simulink model "heatdrive_ecc_coupled_se21"  (R2025b)
settings: Solver=ode23t  StartTime=0.0  StopTime=10  FixedStep=0.1  MaxStep=0.4  RelTol=1e-2  AbsTol=1e-3
values from neighbouring files (symbols this model uses):
  cold_load_heat_W = 0.0    (= 0)    [Build_Simulink_Exchange_Params.m]
  cold_load_T_init = get_stage_field(stage_config, 'cold_load_T_in', get_stage_field(stage_config,          'chip_T_in', get_option_field(exchange_options, 'cold_load_T_init', get_option_field(exchange_options, 'chip_T_init', 293.0))))    [Build_Simulink_Exchange_Params.m]    (also in Create_Simulink_Exchange_Runtime.m = get_option_field(options, 'cold_load_T_init',          get_o)
  cold_sink_T_init = get_stage_field(stage_config, 'cold_sink_T_in', get_option_field(exchange_options, 'cold_sink_T_init', 293.0))    [Build_Simulink_Exchange_Params.m]    (also in Create_Simulink_Exchange_Runtime.m = get_option_field(options, 'cold_sink_T_init', ambient_T_init)
  hot_sink_T_init = get_stage_field(stage_config, 'hot_sink_T_in', get_option_field(exchange_options, 'hot_sink_T_init', 293.0))    [Build_Simulink_Exchange_Params.m]    (also in Create_Simulink_Exchange_Runtime.m = get_option_field(options, 'hot_sink_T_init', ambient_T_init))
  mdot_cooldown_source_kgps = mdot_target_kgps    [Build_Simulink_Exchange_Params.m]
  mdot_hold_source_kgps = mdot_target_kgps    [Build_Simulink_Exchange_Params.m]
  pressure_pi_bias_MPa = pressure_pi_dp_guess_MPa    [Build_Simulink_Exchange_Params.m]
  pressure_pi_error_filter_tau_s = max(get_option_field(exchange_options, 'pressure_pi_error_filter_tau_s', 0.002), 1.0e-5)    [Build_Simulink_Exchange_Params.m]
  pressure_pi_error_normalization_gain_kgps_inv = 1.0    (= 1)    [Build_Simulink_Exchange_Params.m]
  pressure_pi_max_MPa = pressure_pi_dp_guess_MPa + pressure_pi_margin_MPa    [Build_Simulink_Exchange_Params.m]
  shex_sink_T_init = get_option_field(exchange_options, 'shex_sink_T_init', hot_sink_T_init)    [Build_Simulink_Exchange_Params.m]
undefined symbols (not defined in the file or in its folder): constitutive_sample_time_s, constitutive_state21_initial, se_constitutive_T21_initial, se_pressure_integrator_max_MPa, se_pressure_pi_ki_MPa_per_kgps_s, se_pressure_pi_kp_MPa_per_kgps, se_pressure_pi_min_MPa, se_solver_T_init_21_internal, se_stage2_pressure_integrator_min_MPa, se_stage4_pressure_integrator_min_MPa, sma_constitutive_T21_initial, sma_mdot_stage1_source_kgps, sma_mdot_stage3_source_kgps, sma_pressure_integrator_max_MPa, sma_pressure_integrator_min_MPa, sma_pressure_pi_ki_MPa_per_kgps_s, sma_pressure_pi_kp_MPa_per_kgps, sma_pressure_pi_min_MPa, sma_solver_T_init_21_internal
libraries: fl_lib x484, nesl_utility x232, SimscapeFluids_lib x20
(part 7 of 8)

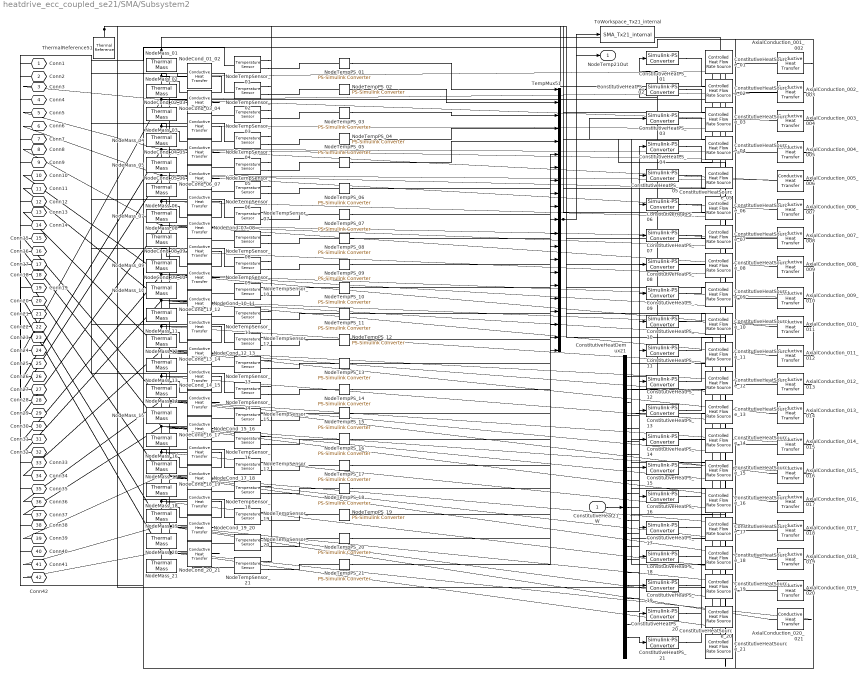
== system heatdrive_ecc_coupled_se21/SMA/Subsystem2 ==
  ConstitutiveHeat21_W : Inport
  AxialConduction_001_002 : fl_lib/Thermal/Thermal Elements/Conductive Heat Transfer  thermal_type=foundation.enum.ConstantVariableTabulated.Constant  wall_geometry=foundation.enum.ConductionWallGeometry.Planar  area=sma_solid_axial_area_m2 m^2  thickness=sma_solid_node_dx_m m  d_in=0.05 m  d_out=0.1 m  L=1 m  th_cond_min=10 W/(K*m)  th_cond=sma_solid_k_W_per_mK W/(K*m)  th_cond_TLU=[413, 401, 392, 383, 371, 357, 342] W/(K*m)  temp_TLU=[200, 273, 400, 600, 800, 1000, 1200] K  T_specify=off  T_priority=None  T=0 K  T_nominal_specify=off  T_nominal_value=1  T_nominal_unit=K  Q_specify=off  Q_priority=None  Q=0 W  Q_nominal_specify=off  Q_nominal_value=1  Q_nominal_unit=W
  AxialConduction_002_003 : fl_lib/Thermal/Thermal Elements/Conductive Heat Transfer  thermal_type=foundation.enum.ConstantVariableTabulated.Constant  wall_geometry=foundation.enum.ConductionWallGeometry.Planar  area=sma_solid_axial_area_m2 m^2  thickness=sma_solid_node_dx_m m  d_in=0.05 m  d_out=0.1 m  L=1 m  th_cond_min=10 W/(K*m)  th_cond=sma_solid_k_W_per_mK W/(K*m)  th_cond_TLU=[413, 401, 392, 383, 371, 357, 342] W/(K*m)  temp_TLU=[200, 273, 400, 600, 800, 1000, 1200] K  T_specify=off  T_priority=None  T=0 K  T_nominal_specify=off  T_nominal_value=1  T_nominal_unit=K  Q_specify=off  Q_priority=None  Q=0 W  Q_nominal_specify=off  Q_nominal_value=1  Q_nominal_unit=W
  AxialConduction_003_004 : fl_lib/Thermal/Thermal Elements/Conductive Heat Transfer  thermal_type=foundation.enum.ConstantVariableTabulated.Constant  wall_geometry=foundation.enum.ConductionWallGeometry.Planar  area=sma_solid_axial_area_m2 m^2  thickness=sma_solid_node_dx_m m  d_in=0.05 m  d_out=0.1 m  L=1 m  th_cond_min=10 W/(K*m)  th_cond=sma_solid_k_W_per_mK W/(K*m)  th_cond_TLU=[413, 401, 392, 383, 371, 357, 342] W/(K*m)  temp_TLU=[200, 273, 400, 600, 800, 1000, 1200] K  T_specify=off  T_priority=None  T=0 K  T_nominal_specify=off  T_nominal_value=1  T_nominal_unit=K  Q_specify=off  Q_priority=None  Q=0 W  Q_nominal_specify=off  Q_nominal_value=1  Q_nominal_unit=W
  AxialConduction_004_005 : fl_lib/Thermal/Thermal Elements/Conductive Heat Transfer  thermal_type=foundation.enum.ConstantVariableTabulated.Constant  wall_geometry=foundation.enum.ConductionWallGeometry.Planar  area=sma_solid_axial_area_m2 m^2  thickness=sma_solid_node_dx_m m  d_in=0.05 m  d_out=0.1 m  L=1 m  th_cond_min=10 W/(K*m)  th_cond=sma_solid_k_W_per_mK W/(K*m)  th_cond_TLU=[413, 401, 392, 383, 371, 357, 342] W/(K*m)  temp_TLU=[200, 273, 400, 600, 800, 1000, 1200] K  T_specify=off  T_priority=None  T=0 K  T_nominal_specify=off  T_nominal_value=1  T_nominal_unit=K  Q_specify=off  Q_priority=None  Q=0 W  Q_nominal_specify=off  Q_nominal_value=1  Q_nominal_unit=W
  AxialConduction_005_006 : fl_lib/Thermal/Thermal Elements/Conductive Heat Transfer  thermal_type=foundation.enum.ConstantVariableTabulated.Constant  wall_geometry=foundation.enum.ConductionWallGeometry.Planar  area=sma_solid_axial_area_m2 m^2  thickness=sma_solid_node_dx_m m  d_in=0.05 m  d_out=0.1 m  L=1 m  th_cond_min=10 W/(K*m)  th_cond=sma_solid_k_W_per_mK W/(K*m)  th_cond_TLU=[413, 401, 392, 383, 371, 357, 342] W/(K*m)  temp_TLU=[200, 273, 400, 600, 800, 1000, 1200] K  T_specify=off  T_priority=None  T=0 K  T_nominal_specify=off  T_nominal_value=1  T_nominal_unit=K  Q_specify=off  Q_priority=None  Q=0 W  Q_nominal_specify=off  Q_nominal_value=1  Q_nominal_unit=W
  AxialConduction_006_007 : fl_lib/Thermal/Thermal Elements/Conductive Heat Transfer  thermal_type=foundation.enum.ConstantVariableTabulated.Constant  wall_geometry=foundation.enum.ConductionWallGeometry.Planar  area=sma_solid_axial_area_m2 m^2  thickness=sma_solid_node_dx_m m  d_in=0.05 m  d_out=0.1 m  L=1 m  th_cond_min=10 W/(K*m)  th_cond=sma_solid_k_W_per_mK W/(K*m)  th_cond_TLU=[413, 401, 392, 383, 371, 357, 342] W/(K*m)  temp_TLU=[200, 273, 400, 600, 800, 1000, 1200] K  T_specify=off  T_priority=None  T=0 K  T_nominal_specify=off  T_nominal_value=1  T_nominal_unit=K  Q_specify=off  Q_priority=None  Q=0 W  Q_nominal_specify=off  Q_nominal_value=1  Q_nominal_unit=W
  AxialConduction_007_008 : fl_lib/Thermal/Thermal Elements/Conductive Heat Transfer  thermal_type=foundation.enum.ConstantVariableTabulated.Constant  wall_geometry=foundation.enum.ConductionWallGeometry.Planar  area=sma_solid_axial_area_m2 m^2  thickness=sma_solid_node_dx_m m  d_in=0.05 m  d_out=0.1 m  L=1 m  th_cond_min=10 W/(K*m)  th_cond=sma_solid_k_W_per_mK W/(K*m)  th_cond_TLU=[413, 401, 392, 383, 371, 357, 342] W/(K*m)  temp_TLU=[200, 273, 400, 600, 800, 1000, 1200] K  T_specify=off  T_priority=None  T=0 K  T_nominal_specify=off  T_nominal_value=1  T_nominal_unit=K  Q_specify=off  Q_priority=None  Q=0 W  Q_nominal_specify=off  Q_nominal_value=1  Q_nominal_unit=W
  AxialConduction_008_009 : fl_lib/Thermal/Thermal Elements/Conductive Heat Transfer  thermal_type=foundation.enum.ConstantVariableTabulated.Constant  wall_geometry=foundation.enum.ConductionWallGeometry.Planar  area=sma_solid_axial_area_m2 m^2  thickness=sma_solid_node_dx_m m  d_in=0.05 m  d_out=0.1 m  L=1 m  th_cond_min=10 W/(K*m)  th_cond=sma_solid_k_W_per_mK W/(K*m)  th_cond_TLU=[413, 401, 392, 383, 371, 357, 342] W/(K*m)  temp_TLU=[200, 273, 400, 600, 800, 1000, 1200] K  T_specify=off  T_priority=None  T=0 K  T_nominal_specify=off  T_nominal_value=1  T_nominal_unit=K  Q_specify=off  Q_priority=None  Q=0 W  Q_nominal_specify=off  Q_nominal_value=1  Q_nominal_unit=W
  AxialConduction_009_010 : fl_lib/Thermal/Thermal Elements/Conductive Heat Transfer  thermal_type=foundation.enum.ConstantVariableTabulated.Constant  wall_geometry=foundation.enum.ConductionWallGeometry.Planar  area=sma_solid_axial_area_m2 m^2  thickness=sma_solid_node_dx_m m  d_in=0.05 m  d_out=0.1 m  L=1 m  th_cond_min=10 W/(K*m)  th_cond=sma_solid_k_W_per_mK W/(K*m)  th_cond_TLU=[413, 401, 392, 383, 371, 357, 342] W/(K*m)  temp_TLU=[200, 273, 400, 600, 800, 1000, 1200] K  T_specify=off  T_priority=None  T=0 K  T_nominal_specify=off  T_nominal_value=1  T_nominal_unit=K  Q_specify=off  Q_priority=None  Q=0 W  Q_nominal_specify=off  Q_nominal_value=1  Q_nominal_unit=W
  AxialConduction_010_011 : fl_lib/Thermal/Thermal Elements/Conductive Heat Transfer  thermal_type=foundation.enum.ConstantVariableTabulated.Constant  wall_geometry=foundation.enum.ConductionWallGeometry.Planar  area=sma_solid_axial_area_m2 m^2  thickness=sma_solid_node_dx_m m  d_in=0.05 m  d_out=0.1 m  L=1 m  th_cond_min=10 W/(K*m)  th_cond=sma_solid_k_W_per_mK W/(K*m)  th_cond_TLU=[413, 401, 392, 383, 371, 357, 342] W/(K*m)  temp_TLU=[200, 273, 400, 600, 800, 1000, 1200] K  T_specify=off  T_priority=None  T=0 K  T_nominal_specify=off  T_nominal_value=1  T_nominal_unit=K  Q_specify=off  Q_priority=None  Q=0 W  Q_nominal_specify=off  Q_nominal_value=1  Q_nominal_unit=W
  AxialConduction_011_012 : fl_lib/Thermal/Thermal Elements/Conductive Heat Transfer  thermal_type=foundation.enum.ConstantVariableTabulated.Constant  wall_geometry=foundation.enum.ConductionWallGeometry.Planar  area=sma_solid_axial_area_m2 m^2  thickness=sma_solid_node_dx_m m  d_in=0.05 m  d_out=0.1 m  L=1 m  th_cond_min=10 W/(K*m)  th_cond=sma_solid_k_W_per_mK W/(K*m)  th_cond_TLU=[413, 401, 392, 383, 371, 357, 342] W/(K*m)  temp_TLU=[200, 273, 400, 600, 800, 1000, 1200] K  T_specify=off  T_priority=None  T=0 K  T_nominal_specify=off  T_nominal_value=1  T_nominal_unit=K  Q_specify=off  Q_priority=None  Q=0 W  Q_nominal_specify=off  Q_nominal_value=1  Q_nominal_unit=W
  AxialConduction_012_013 : fl_lib/Thermal/Thermal Elements/Conductive Heat Transfer  thermal_type=foundation.enum.ConstantVariableTabulated.Constant  wall_geometry=foundation.enum.ConductionWallGeometry.Planar  area=sma_solid_axial_area_m2 m^2  thickness=sma_solid_node_dx_m m  d_in=0.05 m  d_out=0.1 m  L=1 m  th_cond_min=10 W/(K*m)  th_cond=sma_solid_k_W_per_mK W/(K*m)  th_cond_TLU=[413, 401, 392, 383, 371, 357, 342] W/(K*m)  temp_TLU=[200, 273, 400, 600, 800, 1000, 1200] K  T_specify=off  T_priority=None  T=0 K  T_nominal_specify=off  T_nominal_value=1  T_nominal_unit=K  Q_specify=off  Q_priority=None  Q=0 W  Q_nominal_specify=off  Q_nominal_value=1  Q_nominal_unit=W
  AxialConduction_013_014 : fl_lib/Thermal/Thermal Elements/Conductive Heat Transfer  thermal_type=foundation.enum.ConstantVariableTabulated.Constant  wall_geometry=foundation.enum.ConductionWallGeometry.Planar  area=sma_solid_axial_area_m2 m^2  thickness=sma_solid_node_dx_m m  d_in=0.05 m  d_out=0.1 m  L=1 m  th_cond_min=10 W/(K*m)  th_cond=sma_solid_k_W_per_mK W/(K*m)  th_cond_TLU=[413, 401, 392, 383, 371, 357, 342] W/(K*m)  temp_TLU=[200, 273, 400, 600, 800, 1000, 1200] K  T_specify=off  T_priority=None  T=0 K  T_nominal_specify=off  T_nominal_value=1  T_nominal_unit=K  Q_specify=off  Q_priority=None  Q=0 W  Q_nominal_specify=off  Q_nominal_value=1  Q_nominal_unit=W
  AxialConduction_014_015 : fl_lib/Thermal/Thermal Elements/Conductive Heat Transfer  thermal_type=foundation.enum.ConstantVariableTabulated.Constant  wall_geometry=foundation.enum.ConductionWallGeometry.Planar  area=sma_solid_axial_area_m2 m^2  thickness=sma_solid_node_dx_m m  d_in=0.05 m  d_out=0.1 m  L=1 m  th_cond_min=10 W/(K*m)  th_cond=sma_solid_k_W_per_mK W/(K*m)  th_cond_TLU=[413, 401, 392, 383, 371, 357, 342] W/(K*m)  temp_TLU=[200, 273, 400, 600, 800, 1000, 1200] K  T_specify=off  T_priority=None  T=0 K  T_nominal_specify=off  T_nominal_value=1  T_nominal_unit=K  Q_specify=off  Q_priority=None  Q=0 W  Q_nominal_specify=off  Q_nominal_value=1  Q_nominal_unit=W
  AxialConduction_015_016 : fl_lib/Thermal/Thermal Elements/Conductive Heat Transfer  thermal_type=foundation.enum.ConstantVariableTabulated.Constant  wall_geometry=foundation.enum.ConductionWallGeometry.Planar  area=sma_solid_axial_area_m2 m^2  thickness=sma_solid_node_dx_m m  d_in=0.05 m  d_out=0.1 m  L=1 m  th_cond_min=10 W/(K*m)  th_cond=sma_solid_k_W_per_mK W/(K*m)  th_cond_TLU=[413, 401, 392, 383, 371, 357, 342] W/(K*m)  temp_TLU=[200, 273, 400, 600, 800, 1000, 1200] K  T_specify=off  T_priority=None  T=0 K  T_nominal_specify=off  T_nominal_value=1  T_nominal_unit=K  Q_specify=off  Q_priority=None  Q=0 W  Q_nominal_specify=off  Q_nominal_value=1  Q_nominal_unit=W
  AxialConduction_016_017 : fl_lib/Thermal/Thermal Elements/Conductive Heat Transfer  thermal_type=foundation.enum.ConstantVariableTabulated.Constant  wall_geometry=foundation.enum.ConductionWallGeometry.Planar  area=sma_solid_axial_area_m2 m^2  thickness=sma_solid_node_dx_m m  d_in=0.05 m  d_out=0.1 m  L=1 m  th_cond_min=10 W/(K*m)  th_cond=sma_solid_k_W_per_mK W/(K*m)  th_cond_TLU=[413, 401, 392, 383, 371, 357, 342] W/(K*m)  temp_TLU=[200, 273, 400, 600, 800, 1000, 1200] K  T_specify=off  T_priority=None  T=0 K  T_nominal_specify=off  T_nominal_value=1  T_nominal_unit=K  Q_specify=off  Q_priority=None  Q=0 W  Q_nominal_specify=off  Q_nominal_value=1  Q_nominal_unit=W
  AxialConduction_017_018 : fl_lib/Thermal/Thermal Elements/Conductive Heat Transfer  thermal_type=foundation.enum.ConstantVariableTabulated.Constant  wall_geometry=foundation.enum.ConductionWallGeometry.Planar  area=sma_solid_axial_area_m2 m^2  thickness=sma_solid_node_dx_m m  d_in=0.05 m  d_out=0.1 m  L=1 m  th_cond_min=10 W/(K*m)  th_cond=sma_solid_k_W_per_mK W/(K*m)  th_cond_TLU=[413, 401, 392, 383, 371, 357, 342] W/(K*m)  temp_TLU=[200, 273, 400, 600, 800, 1000, 1200] K  T_specify=off  T_priority=None  T=0 K  T_nominal_specify=off  T_nominal_value=1  T_nominal_unit=K  Q_specify=off  Q_priority=None  Q=0 W  Q_nominal_specify=off  Q_nominal_value=1  Q_nominal_unit=W
  AxialConduction_018_019 : fl_lib/Thermal/Thermal Elements/Conductive Heat Transfer  thermal_type=foundation.enum.ConstantVariableTabulated.Constant  wall_geometry=foundation.enum.ConductionWallGeometry.Planar  area=sma_solid_axial_area_m2 m^2  thickness=sma_solid_node_dx_m m  d_in=0.05 m  d_out=0.1 m  L=1 m  th_cond_min=10 W/(K*m)  th_cond=sma_solid_k_W_per_mK W/(K*m)  th_cond_TLU=[413, 401, 392, 383, 371, 357, 342] W/(K*m)  temp_TLU=[200, 273, 400, 600, 800, 1000, 1200] K  T_specify=off  T_priority=None  T=0 K  T_nominal_specify=off  T_nominal_value=1  T_nominal_unit=K  Q_specify=off  Q_priority=None  Q=0 W  Q_nominal_specify=off  Q_nominal_value=1  Q_nominal_unit=W
  AxialConduction_019_020 : fl_lib/Thermal/Thermal Elements/Conductive Heat Transfer  thermal_type=foundation.enum.ConstantVariableTabulated.Constant  wall_geometry=foundation.enum.ConductionWallGeometry.Planar  area=sma_solid_axial_area_m2 m^2  thickness=sma_solid_node_dx_m m  d_in=0.05 m  d_out=0.1 m  L=1 m  th_cond_min=10 W/(K*m)  th_cond=sma_solid_k_W_per_mK W/(K*m)  th_cond_TLU=[413, 401, 392, 383, 371, 357, 342] W/(K*m)  temp_TLU=[200, 273, 400, 600, 800, 1000, 1200] K  T_specify=off  T_priority=None  T=0 K  T_nominal_specify=off  T_nominal_value=1  T_nominal_unit=K  Q_specify=off  Q_priority=None  Q=0 W  Q_nominal_specify=off  Q_nominal_value=1  Q_nominal_unit=W
  AxialConduction_020_021 : fl_lib/Thermal/Thermal Elements/Conductive Heat Transfer  thermal_type=foundation.enum.ConstantVariableTabulated.Constant  wall_geometry=foundation.enum.ConductionWallGeometry.Planar  area=sma_solid_axial_area_m2 m^2  thickness=sma_solid_node_dx_m m  d_in=0.05 m  d_out=0.1 m  L=1 m  th_cond_min=10 W/(K*m)  th_cond=sma_solid_k_W_per_mK W/(K*m)  th_cond_TLU=[413, 401, 392, 383, 371, 357, 342] W/(K*m)  temp_TLU=[200, 273, 400, 600, 800, 1000, 1200] K  T_specify=off  T_priority=None  T=0 K  T_nominal_specify=off  T_nominal_value=1  T_nominal_unit=K  Q_specify=off  Q_priority=None  Q=0 W  Q_nominal_specify=off  Q_nominal_value=1  Q_nominal_unit=W
  ConstitutiveHeatDemux21 : Demux  Outputs=21
  ConstitutiveHeatPS_01 : nesl_utility/Simulink-PS Converter  PhysicalDomain=network_engine_domain  SubClassName=ps_input  LeftPortType=input  RightPortType=output  PseudoPeriodic=off  Frequencies=[]  NoiseDistribution=none  NoiseParameters=[]  Unit=W  AffineConversion=off  FilteringAndDerivatives=provide  SimscapeFilterOrder=1  InputFilterTimeConstant=0.001  UdotUserProvided=0
  ConstitutiveHeatPS_02 : nesl_utility/Simulink-PS Converter  PhysicalDomain=network_engine_domain  SubClassName=ps_input  LeftPortType=input  RightPortType=output  PseudoPeriodic=off  Frequencies=[]  NoiseDistribution=none  NoiseParameters=[]  Unit=W  AffineConversion=off  FilteringAndDerivatives=provide  SimscapeFilterOrder=1  InputFilterTimeConstant=0.001  UdotUserProvided=0
  ConstitutiveHeatPS_03 : nesl_utility/Simulink-PS Converter  PhysicalDomain=network_engine_domain  SubClassName=ps_input  LeftPortType=input  RightPortType=output  PseudoPeriodic=off  Frequencies=[]  NoiseDistribution=none  NoiseParameters=[]  Unit=W  AffineConversion=off  FilteringAndDerivatives=provide  SimscapeFilterOrder=1  InputFilterTimeConstant=0.001  UdotUserProvided=0
  ConstitutiveHeatPS_04 : nesl_utility/Simulink-PS Converter  PhysicalDomain=network_engine_domain  SubClassName=ps_input  LeftPortType=input  RightPortType=output  PseudoPeriodic=off  Frequencies=[]  NoiseDistribution=none  NoiseParameters=[]  Unit=W  AffineConversion=off  FilteringAndDerivatives=provide  SimscapeFilterOrder=1  InputFilterTimeConstant=0.001  UdotUserProvided=0
  ConstitutiveHeatPS_05 : nesl_utility/Simulink-PS Converter  PhysicalDomain=network_engine_domain  SubClassName=ps_input  LeftPortType=input  RightPortType=output  PseudoPeriodic=off  Frequencies=[]  NoiseDistribution=none  NoiseParameters=[]  Unit=W  AffineConversion=off  FilteringAndDerivatives=provide  SimscapeFilterOrder=1  InputFilterTimeConstant=0.001  UdotUserProvided=0
  ConstitutiveHeatPS_06 : nesl_utility/Simulink-PS Converter  PhysicalDomain=network_engine_domain  SubClassName=ps_input  LeftPortType=input  RightPortType=output  PseudoPeriodic=off  Frequencies=[]  NoiseDistribution=none  NoiseParameters=[]  Unit=W  AffineConversion=off  FilteringAndDerivatives=provide  SimscapeFilterOrder=1  InputFilterTimeConstant=0.001  UdotUserProvided=0
  ConstitutiveHeatPS_07 : nesl_utility/Simulink-PS Converter  PhysicalDomain=network_engine_domain  SubClassName=ps_input  LeftPortType=input  RightPortType=output  PseudoPeriodic=off  Frequencies=[]  NoiseDistribution=none  NoiseParameters=[]  Unit=W  AffineConversion=off  FilteringAndDerivatives=provide  SimscapeFilterOrder=1  InputFilterTimeConstant=0.001  UdotUserProvided=0
  ConstitutiveHeatPS_08 : nesl_utility/Simulink-PS Converter  PhysicalDomain=network_engine_domain  SubClassName=ps_input  LeftPortType=input  RightPortType=output  PseudoPeriodic=off  Frequencies=[]  NoiseDistribution=none  NoiseParameters=[]  Unit=W  AffineConversion=off  FilteringAndDerivatives=provide  SimscapeFilterOrder=1  InputFilterTimeConstant=0.001  UdotUserProvided=0
  ConstitutiveHeatPS_09 : nesl_utility/Simulink-PS Converter  PhysicalDomain=network_engine_domain  SubClassName=ps_input  LeftPortType=input  RightPortType=output  PseudoPeriodic=off  Frequencies=[]  NoiseDistribution=none  NoiseParameters=[]  Unit=W  AffineConversion=off  FilteringAndDerivatives=provide  SimscapeFilterOrder=1  InputFilterTimeConstant=0.001  UdotUserProvided=0
  ConstitutiveHeatPS_{10..21} (12 alike) : nesl_utility/Simulink-PS Converter  PhysicalDomain=network_engine_domain  SubClassName=ps_input  LeftPortType=input  RightPortType=output  PseudoPeriodic=off  Frequencies=[]  NoiseDistribution=none  NoiseParameters=[]  Unit=W  AffineConversion=off  FilteringAndDerivatives=provide  SimscapeFilterOrder=1  InputFilterTimeConstant=0.001  UdotUserProvided=0
  ConstitutiveHeatSource_01 : fl_lib/Thermal/Thermal Sources/Controlled Heat Flow Rate Source
  ConstitutiveHeatSource_02 : fl_lib/Thermal/Thermal Sources/Controlled Heat Flow Rate Source
  ConstitutiveHeatSource_03 : fl_lib/Thermal/Thermal Sources/Controlled Heat Flow Rate Source
  ConstitutiveHeatSource_04 : fl_lib/Thermal/Thermal Sources/Controlled Heat Flow Rate Source
  ConstitutiveHeatSource_05 : fl_lib/Thermal/Thermal Sources/Controlled Heat Flow Rate Source
  ConstitutiveHeatSource_06 : fl_lib/Thermal/Thermal Sources/Controlled Heat Flow Rate Source
  ConstitutiveHeatSource_07 : fl_lib/Thermal/Thermal Sources/Controlled Heat Flow Rate Source
  ConstitutiveHeatSource_08 : fl_lib/Thermal/Thermal Sources/Controlled Heat Flow Rate Source
  ConstitutiveHeatSource_09 : fl_lib/Thermal/Thermal Sources/Controlled Heat Flow Rate Source
  ConstitutiveHeatSource_{10..21} (12 alike) : fl_lib/Thermal/Thermal Sources/Controlled Heat Flow Rate Source
  NodeCond_01_02 : fl_lib/Thermal/Thermal Elements/Conductive Heat Transfer  thermal_type=foundation.enum.ConstantVariableTabulated.Constant  wall_geometry=foundation.enum.ConductionWallGeometry.Planar  area=sma_pipe_fa m^2  thickness=solver51_cond_dx m  d_in=0.05 m  d_out=0.1 m  L=1 m  th_cond_min=10 W/(K*m)  th_cond=solver51_cond_k W/(K*m)  th_cond_TLU=[413, 401, 392, 383, 371, 357, 342] W/(K*m)  temp_TLU=[200, 273, 400, 600, 800, 1000, 1200] K  T_specify=off  T_priority=None  T=0 K  T_nominal_specify=off  T_nominal_value=1  T_nominal_unit=K  Q_specify=off  Q_priority=None  Q=0 W  Q_nominal_specify=off  Q_nominal_value=1  Q_nominal_unit=W
  NodeCond_02_03 : fl_lib/Thermal/Thermal Elements/Conductive Heat Transfer  thermal_type=foundation.enum.ConstantVariableTabulated.Constant  wall_geometry=foundation.enum.ConductionWallGeometry.Planar  area=sma_pipe_fa m^2  thickness=solver51_cond_dx m  d_in=0.05 m  d_out=0.1 m  L=1 m  th_cond_min=10 W/(K*m)  th_cond=solver51_cond_k W/(K*m)  th_cond_TLU=[413, 401, 392, 383, 371, 357, 342] W/(K*m)  temp_TLU=[200, 273, 400, 600, 800, 1000, 1200] K  T_specify=off  T_priority=None  T=0 K  T_nominal_specify=off  T_nominal_value=1  T_nominal_unit=K  Q_specify=off  Q_priority=None  Q=0 W  Q_nominal_specify=off  Q_nominal_value=1  Q_nominal_unit=W
  NodeCond_03_04 : fl_lib/Thermal/Thermal Elements/Conductive Heat Transfer  thermal_type=foundation.enum.ConstantVariableTabulated.Constant  wall_geometry=foundation.enum.ConductionWallGeometry.Planar  area=sma_pipe_fa m^2  thickness=solver51_cond_dx m  d_in=0.05 m  d_out=0.1 m  L=1 m  th_cond_min=10 W/(K*m)  th_cond=solver51_cond_k W/(K*m)  th_cond_TLU=[413, 401, 392, 383, 371, 357, 342] W/(K*m)  temp_TLU=[200, 273, 400, 600, 800, 1000, 1200] K  T_specify=off  T_priority=None  T=0 K  T_nominal_specify=off  T_nominal_value=1  T_nominal_unit=K  Q_specify=off  Q_priority=None  Q=0 W  Q_nominal_specify=off  Q_nominal_value=1  Q_nominal_unit=W
  NodeCond_04_05 : fl_lib/Thermal/Thermal Elements/Conductive Heat Transfer  thermal_type=foundation.enum.ConstantVariableTabulated.Constant  wall_geometry=foundation.enum.ConductionWallGeometry.Planar  area=sma_pipe_fa m^2  thickness=solver51_cond_dx m  d_in=0.05 m  d_out=0.1 m  L=1 m  th_cond_min=10 W/(K*m)  th_cond=solver51_cond_k W/(K*m)  th_cond_TLU=[413, 401, 392, 383, 371, 357, 342] W/(K*m)  temp_TLU=[200, 273, 400, 600, 800, 1000, 1200] K  T_specify=off  T_priority=None  T=0 K  T_nominal_specify=off  T_nominal_value=1  T_nominal_unit=K  Q_specify=off  Q_priority=None  Q=0 W  Q_nominal_specify=off  Q_nominal_value=1  Q_nominal_unit=W
  NodeCond_05_06 : fl_lib/Thermal/Thermal Elements/Conductive Heat Transfer  thermal_type=foundation.enum.ConstantVariableTabulated.Constant  wall_geometry=foundation.enum.ConductionWallGeometry.Planar  area=sma_pipe_fa m^2  thickness=solver51_cond_dx m  d_in=0.05 m  d_out=0.1 m  L=1 m  th_cond_min=10 W/(K*m)  th_cond=solver51_cond_k W/(K*m)  th_cond_TLU=[413, 401, 392, 383, 371, 357, 342] W/(K*m)  temp_TLU=[200, 273, 400, 600, 800, 1000, 1200] K  T_specify=off  T_priority=None  T=0 K  T_nominal_specify=off  T_nominal_value=1  T_nominal_unit=K  Q_specify=off  Q_priority=None  Q=0 W  Q_nominal_specify=off  Q_nominal_value=1  Q_nominal_unit=W
  NodeCond_06_07 : fl_lib/Thermal/Thermal Elements/Conductive Heat Transfer  thermal_type=foundation.enum.ConstantVariableTabulated.Constant  wall_geometry=foundation.enum.ConductionWallGeometry.Planar  area=sma_pipe_fa m^2  thickness=solver51_cond_dx m  d_in=0.05 m  d_out=0.1 m  L=1 m  th_cond_min=10 W/(K*m)  th_cond=solver51_cond_k W/(K*m)  th_cond_TLU=[413, 401, 392, 383, 371, 357, 342] W/(K*m)  temp_TLU=[200, 273, 400, 600, 800, 1000, 1200] K  T_specify=off  T_priority=None  T=0 K  T_nominal_specify=off  T_nominal_value=1  T_nominal_unit=K  Q_specify=off  Q_priority=None  Q=0 W  Q_nominal_specify=off  Q_nominal_value=1  Q_nominal_unit=W
  NodeCond_07_08 : fl_lib/Thermal/Thermal Elements/Conductive Heat Transfer  thermal_type=foundation.enum.ConstantVariableTabulated.Constant  wall_geometry=foundation.enum.ConductionWallGeometry.Planar  area=sma_pipe_fa m^2  thickness=solver51_cond_dx m  d_in=0.05 m  d_out=0.1 m  L=1 m  th_cond_min=10 W/(K*m)  th_cond=solver51_cond_k W/(K*m)  th_cond_TLU=[413, 401, 392, 383, 371, 357, 342] W/(K*m)  temp_TLU=[200, 273, 400, 600, 800, 1000, 1200] K  T_specify=off  T_priority=None  T=0 K  T_nominal_specify=off  T_nominal_value=1  T_nominal_unit=K  Q_specify=off  Q_priority=None  Q=0 W  Q_nominal_specify=off  Q_nominal_value=1  Q_nominal_unit=W
  NodeCond_08_09 : fl_lib/Thermal/Thermal Elements/Conductive Heat Transfer  thermal_type=foundation.enum.ConstantVariableTabulated.Constant  wall_geometry=foundation.enum.ConductionWallGeometry.Planar  area=sma_pipe_fa m^2  thickness=solver51_cond_dx m  d_in=0.05 m  d_out=0.1 m  L=1 m  th_cond_min=10 W/(K*m)  th_cond=solver51_cond_k W/(K*m)  th_cond_TLU=[413, 401, 392, 383, 371, 357, 342] W/(K*m)  temp_TLU=[200, 273, 400, 600, 800, 1000, 1200] K  T_specify=off  T_priority=None  T=0 K  T_nominal_specify=off  T_nominal_value=1  T_nominal_unit=K  Q_specify=off  Q_priority=None  Q=0 W  Q_nominal_specify=off  Q_nominal_value=1  Q_nominal_unit=W
  NodeCond_09_10 : fl_lib/Thermal/Thermal Elements/Conductive Heat Transfer  thermal_type=foundation.enum.ConstantVariableTabulated.Constant  wall_geometry=foundation.enum.ConductionWallGeometry.Planar  area=sma_pipe_fa m^2  thickness=solver51_cond_dx m  d_in=0.05 m  d_out=0.1 m  L=1 m  th_cond_min=10 W/(K*m)  th_cond=solver51_cond_k W/(K*m)  th_cond_TLU=[413, 401, 392, 383, 371, 357, 342] W/(K*m)  temp_TLU=[200, 273, 400, 600, 800, 1000, 1200] K  T_specify=off  T_priority=None  T=0 K  T_nominal_specify=off  T_nominal_value=1  T_nominal_unit=K  Q_specify=off  Q_priority=None  Q=0 W  Q_nominal_specify=off  Q_nominal_value=1  Q_nominal_unit=W
  NodeCond_10_11 : fl_lib/Thermal/Thermal Elements/Conductive Heat Transfer  thermal_type=foundation.enum.ConstantVariableTabulated.Constant  wall_geometry=foundation.enum.ConductionWallGeometry.Planar  area=sma_pipe_fa m^2  thickness=solver51_cond_dx m  d_in=0.05 m  d_out=0.1 m  L=1 m  th_cond_min=10 W/(K*m)  th_cond=solver51_cond_k W/(K*m)  th_cond_TLU=[413, 401, 392, 383, 371, 357, 342] W/(K*m)  temp_TLU=[200, 273, 400, 600, 800, 1000, 1200] K  T_specify=off  T_priority=None  T=0 K  T_nominal_specify=off  T_nominal_value=1  T_nominal_unit=K  Q_specify=off  Q_priority=None  Q=0 W  Q_nominal_specify=off  Q_nominal_value=1  Q_nominal_unit=W
  NodeCond_11_12 : fl_lib/Thermal/Thermal Elements/Conductive Heat Transfer  thermal_type=foundation.enum.ConstantVariableTabulated.Constant  wall_geometry=foundation.enum.ConductionWallGeometry.Planar  area=sma_pipe_fa m^2  thickness=solver51_cond_dx m  d_in=0.05 m  d_out=0.1 m  L=1 m  th_cond_min=10 W/(K*m)  th_cond=solver51_cond_k W/(K*m)  th_cond_TLU=[413, 401, 392, 383, 371, 357, 342] W/(K*m)  temp_TLU=[200, 273, 400, 600, 800, 1000, 1200] K  T_specify=off  T_priority=None  T=0 K  T_nominal_specify=off  T_nominal_value=1  T_nominal_unit=K  Q_specify=off  Q_priority=None  Q=0 W  Q_nominal_specify=off  Q_nominal_value=1  Q_nominal_unit=W
  NodeCond_12_13 : fl_lib/Thermal/Thermal Elements/Conductive Heat Transfer  thermal_type=foundation.enum.ConstantVariableTabulated.Constant  wall_geometry=foundation.enum.ConductionWallGeometry.Planar  area=sma_pipe_fa m^2  thickness=solver51_cond_dx m  d_in=0.05 m  d_out=0.1 m  L=1 m  th_cond_min=10 W/(K*m)  th_cond=solver51_cond_k W/(K*m)  th_cond_TLU=[413, 401, 392, 383, 371, 357, 342] W/(K*m)  temp_TLU=[200, 273, 400, 600, 800, 1000, 1200] K  T_specify=off  T_priority=None  T=0 K  T_nominal_specify=off  T_nominal_value=1  T_nominal_unit=K  Q_specify=off  Q_priority=None  Q=0 W  Q_nominal_specify=off  Q_nominal_value=1  Q_nominal_unit=W
  NodeCond_13_14 : fl_lib/Thermal/Thermal Elements/Conductive Heat Transfer  thermal_type=foundation.enum.ConstantVariableTabulated.Constant  wall_geometry=foundation.enum.ConductionWallGeometry.Planar  area=sma_pipe_fa m^2  thickness=solver51_cond_dx m  d_in=0.05 m  d_out=0.1 m  L=1 m  th_cond_min=10 W/(K*m)  th_cond=solver51_cond_k W/(K*m)  th_cond_TLU=[413, 401, 392, 383, 371, 357, 342] W/(K*m)  temp_TLU=[200, 273, 400, 600, 800, 1000, 1200] K  T_specify=off  T_priority=None  T=0 K  T_nominal_specify=off  T_nominal_value=1  T_nominal_unit=K  Q_specify=off  Q_priority=None  Q=0 W  Q_nominal_specify=off  Q_nominal_value=1  Q_nominal_unit=W
  NodeCond_14_15 : fl_lib/Thermal/Thermal Elements/Conductive Heat Transfer  thermal_type=foundation.enum.ConstantVariableTabulated.Constant  wall_geometry=foundation.enum.ConductionWallGeometry.Planar  area=sma_pipe_fa m^2  thickness=solver51_cond_dx m  d_in=0.05 m  d_out=0.1 m  L=1 m  th_cond_min=10 W/(K*m)  th_cond=solver51_cond_k W/(K*m)  th_cond_TLU=[413, 401, 392, 383, 371, 357, 342] W/(K*m)  temp_TLU=[200, 273, 400, 600, 800, 1000, 1200] K  T_specify=off  T_priority=None  T=0 K  T_nominal_specify=off  T_nominal_value=1  T_nominal_unit=K  Q_specify=off  Q_priority=None  Q=0 W  Q_nominal_specify=off  Q_nominal_value=1  Q_nominal_unit=W
  NodeCond_15_16 : fl_lib/Thermal/Thermal Elements/Conductive Heat Transfer  thermal_type=foundation.enum.ConstantVariableTabulated.Constant  wall_geometry=foundation.enum.ConductionWallGeometry.Planar  area=sma_pipe_fa m^2  thickness=solver51_cond_dx m  d_in=0.05 m  d_out=0.1 m  L=1 m  th_cond_min=10 W/(K*m)  th_cond=solver51_cond_k W/(K*m)  th_cond_TLU=[413, 401, 392, 383, 371, 357, 342] W/(K*m)  temp_TLU=[200, 273, 400, 600, 800, 1000, 1200] K  T_specify=off  T_priority=None  T=0 K  T_nominal_specify=off  T_nominal_value=1  T_nominal_unit=K  Q_specify=off  Q_priority=None  Q=0 W  Q_nominal_specify=off  Q_nominal_value=1  Q_nominal_unit=W
  NodeCond_16_17 : fl_lib/Thermal/Thermal Elements/Conductive Heat Transfer  thermal_type=foundation.enum.ConstantVariableTabulated.Constant  wall_geometry=foundation.enum.ConductionWallGeometry.Planar  area=sma_pipe_fa m^2  thickness=solver51_cond_dx m  d_in=0.05 m  d_out=0.1 m  L=1 m  th_cond_min=10 W/(K*m)  th_cond=solver51_cond_k W/(K*m)  th_cond_TLU=[413, 401, 392, 383, 371, 357, 342] W/(K*m)  temp_TLU=[200, 273, 400, 600, 800, 1000, 1200] K  T_specify=off  T_priority=None  T=0 K  T_nominal_specify=off  T_nominal_value=1  T_nominal_unit=K  Q_specify=off  Q_priority=None  Q=0 W  Q_nominal_specify=off  Q_nominal_value=1  Q_nominal_unit=W
  NodeCond_17_18 : fl_lib/Thermal/Thermal Elements/Conductive Heat Transfer  thermal_type=foundation.enum.ConstantVariableTabulated.Constant  wall_geometry=foundation.enum.ConductionWallGeometry.Planar  area=sma_pipe_fa m^2  thickness=solver51_cond_dx m  d_in=0.05 m  d_out=0.1 m  L=1 m  th_cond_min=10 W/(K*m)  th_cond=solver51_cond_k W/(K*m)  th_cond_TLU=[413, 401, 392, 383, 371, 357, 342] W/(K*m)  temp_TLU=[200, 273, 400, 600, 800, 1000, 1200] K  T_specify=off  T_priority=None  T=0 K  T_nominal_specify=off  T_nominal_value=1  T_nominal_unit=K  Q_specify=off  Q_priority=None  Q=0 W  Q_nominal_specify=off  Q_nominal_value=1  Q_nominal_unit=W
  NodeCond_18_19 : fl_lib/Thermal/Thermal Elements/Conductive Heat Transfer  thermal_type=foundation.enum.ConstantVariableTabulated.Constant  wall_geometry=foundation.enum.ConductionWallGeometry.Planar  area=sma_pipe_fa m^2  thickness=solver51_cond_dx m  d_in=0.05 m  d_out=0.1 m  L=1 m  th_cond_min=10 W/(K*m)  th_cond=solver51_cond_k W/(K*m)  th_cond_TLU=[413, 401, 392, 383, 371, 357, 342] W/(K*m)  temp_TLU=[200, 273, 400, 600, 800, 1000, 1200] K  T_specify=off  T_priority=None  T=0 K  T_nominal_specify=off  T_nominal_value=1  T_nominal_unit=K  Q_specify=off  Q_priority=None  Q=0 W  Q_nominal_specify=off  Q_nominal_value=1  Q_nominal_unit=W
  NodeCond_19_20 : fl_lib/Thermal/Thermal Elements/Conductive Heat Transfer  thermal_type=foundation.enum.ConstantVariableTabulated.Constant  wall_geometry=foundation.enum.ConductionWallGeometry.Planar  area=sma_pipe_fa m^2  thickness=solver51_cond_dx m  d_in=0.05 m  d_out=0.1 m  L=1 m  th_cond_min=10 W/(K*m)  th_cond=solver51_cond_k W/(K*m)  th_cond_TLU=[413, 401, 392, 383, 371, 357, 342] W/(K*m)  temp_TLU=[200, 273, 400, 600, 800, 1000, 1200] K  T_specify=off  T_priority=None  T=0 K  T_nominal_specify=off  T_nominal_value=1  T_nominal_unit=K  Q_specify=off  Q_priority=None  Q=0 W  Q_nominal_specify=off  Q_nominal_value=1  Q_nominal_unit=W
  NodeCond_20_21 : fl_lib/Thermal/Thermal Elements/Conductive Heat Transfer  thermal_type=foundation.enum.ConstantVariableTabulated.Constant  wall_geometry=foundation.enum.ConductionWallGeometry.Planar  area=sma_pipe_fa m^2  thickness=solver51_cond_dx m  d_in=0.05 m  d_out=0.1 m  L=1 m  th_cond_min=10 W/(K*m)  th_cond=solver51_cond_k W/(K*m)  th_cond_TLU=[413, 401, 392, 383, 371, 357, 342] W/(K*m)  temp_TLU=[200, 273, 400, 600, 800, 1000, 1200] K  T_specify=off  T_priority=None  T=0 K  T_nominal_specify=off  T_nominal_value=1  T_nominal_unit=K  Q_specify=off  Q_priority=None  Q=0 W  Q_nominal_specify=off  Q_nominal_value=1  Q_nominal_unit=W
  NodeMass_01 : fl_lib/Thermal/Thermal Elements/Thermal Mass  mass_type=foundation.enum.constant_variable.constant  mass=sma_node_mass_kg kg  sp_heat=sma_node_cp J/(K*kg)  mass_min=1e-6 kg  num_ports=foundation.enum.numPorts2.one  m_specify=off  m_priority=High  m=1 kg  m_nominal_specify=off  m_nominal_value=1  m_nominal_unit=kg  T_specify=on  T_priority=High  T=sma_solver_T_init_21_internal(1) K  T_nominal_specify=off  T_nominal_value=1  T_nominal_unit=K  Q_specify=off  Q_priority=None  Q=0 W  Q_nominal_specify=off  Q_nominal_value=1  Q_nominal_unit=W
  NodeMass_02 : fl_lib/Thermal/Thermal Elements/Thermal Mass  mass_type=foundation.enum.constant_variable.constant  mass=sma_node_mass_kg kg  sp_heat=sma_node_cp J/(K*kg)  mass_min=1e-6 kg  num_ports=foundation.enum.numPorts2.one  m_specify=off  m_priority=High  m=1 kg  m_nominal_specify=off  m_nominal_value=1  m_nominal_unit=kg  T_specify=on  T_priority=High  T=sma_solver_T_init_21_internal(2) K  T_nominal_specify=off  T_nominal_value=1  T_nominal_unit=K  Q_specify=off  Q_priority=None  Q=0 W  Q_nominal_specify=off  Q_nominal_value=1  Q_nominal_unit=W
  NodeMass_03 : fl_lib/Thermal/Thermal Elements/Thermal Mass  mass_type=foundation.enum.constant_variable.constant  mass=sma_node_mass_kg kg  sp_heat=sma_node_cp J/(K*kg)  mass_min=1e-6 kg  num_ports=foundation.enum.numPorts2.one  m_specify=off  m_priority=High  m=1 kg  m_nominal_specify=off  m_nominal_value=1  m_nominal_unit=kg  T_specify=on  T_priority=High  T=sma_solver_T_init_21_internal(3) K  T_nominal_specify=off  T_nominal_value=1  T_nominal_unit=K  Q_specify=off  Q_priority=None  Q=0 W  Q_nominal_specify=off  Q_nominal_value=1  Q_nominal_unit=W
  NodeMass_04 : fl_lib/Thermal/Thermal Elements/Thermal Mass  mass_type=foundation.enum.constant_variable.constant  mass=sma_node_mass_kg kg  sp_heat=sma_node_cp J/(K*kg)  mass_min=1e-6 kg  num_ports=foundation.enum.numPorts2.one  m_specify=off  m_priority=High  m=1 kg  m_nominal_specify=off  m_nominal_value=1  m_nominal_unit=kg  T_specify=on  T_priority=High  T=sma_solver_T_init_21_internal(4) K  T_nominal_specify=off  T_nominal_value=1  T_nominal_unit=K  Q_specify=off  Q_priority=None  Q=0 W  Q_nominal_specify=off  Q_nominal_value=1  Q_nominal_unit=W
  NodeMass_05 : fl_lib/Thermal/Thermal Elements/Thermal Mass  mass_type=foundation.enum.constant_variable.constant  mass=sma_node_mass_kg kg  sp_heat=sma_node_cp J/(K*kg)  mass_min=1e-6 kg  num_ports=foundation.enum.numPorts2.one  m_specify=off  m_priority=High  m=1 kg  m_nominal_specify=off  m_nominal_value=1  m_nominal_unit=kg  T_specify=on  T_priority=High  T=sma_solver_T_init_21_internal(5) K  T_nominal_specify=off  T_nominal_value=1  T_nominal_unit=K  Q_specify=off  Q_priority=None  Q=0 W  Q_nominal_specify=off  Q_nominal_value=1  Q_nominal_unit=W
  NodeMass_06 : fl_lib/Thermal/Thermal Elements/Thermal Mass  mass_type=foundation.enum.constant_variable.constant  mass=sma_node_mass_kg kg  sp_heat=sma_node_cp J/(K*kg)  mass_min=1e-6 kg  num_ports=foundation.enum.numPorts2.one  m_specify=off  m_priority=High  m=1 kg  m_nominal_specify=off  m_nominal_value=1  m_nominal_unit=kg  T_specify=on  T_priority=High  T=sma_solver_T_init_21_internal(6) K  T_nominal_specify=off  T_nominal_value=1  T_nominal_unit=K  Q_specify=off  Q_priority=None  Q=0 W  Q_nominal_specify=off  Q_nominal_value=1  Q_nominal_unit=W
  NodeMass_07 : fl_lib/Thermal/Thermal Elements/Thermal Mass  mass_type=foundation.enum.constant_variable.constant  mass=sma_node_mass_kg kg  sp_heat=sma_node_cp J/(K*kg)  mass_min=1e-6 kg  num_ports=foundation.enum.numPorts2.one  m_specify=off  m_priority=High  m=1 kg  m_nominal_specify=off  m_nominal_value=1  m_nominal_unit=kg  T_specify=on  T_priority=High  T=sma_solver_T_init_21_internal(7) K  T_nominal_specify=off  T_nominal_value=1  T_nominal_unit=K  Q_specify=off  Q_priority=None  Q=0 W  Q_nominal_specify=off  Q_nominal_value=1  Q_nominal_unit=W
  NodeMass_08 : fl_lib/Thermal/Thermal Elements/Thermal Mass  mass_type=foundation.enum.constant_variable.constant  mass=sma_node_mass_kg kg  sp_heat=sma_node_cp J/(K*kg)  mass_min=1e-6 kg  num_ports=foundation.enum.numPorts2.one  m_specify=off  m_priority=High  m=1 kg  m_nominal_specify=off  m_nominal_value=1  m_nominal_unit=kg  T_specify=on  T_priority=High  T=sma_solver_T_init_21_internal(8) K  T_nominal_specify=off  T_nominal_value=1  T_nominal_unit=K  Q_specify=off  Q_priority=None  Q=0 W  Q_nominal_specify=off  Q_nominal_value=1  Q_nominal_unit=W
  NodeMass_09 : fl_lib/Thermal/Thermal Elements/Thermal Mass  mass_type=foundation.enum.constant_variable.constant  mass=sma_node_mass_kg kg  sp_heat=sma_node_cp J/(K*kg)  mass_min=1e-6 kg  num_ports=foundation.enum.numPorts2.one  m_specify=off  m_priority=High  m=1 kg  m_nominal_specify=off  m_nominal_value=1  m_nominal_unit=kg  T_specify=on  T_priority=High  T=sma_solver_T_init_21_internal(9) K  T_nominal_specify=off  T_nominal_value=1  T_nominal_unit=K  Q_specify=off  Q_priority=None  Q=0 W  Q_nominal_specify=off  Q_nominal_value=1  Q_nominal_unit=W
  NodeMass_10 : fl_lib/Thermal/Thermal Elements/Thermal Mass  mass_type=foundation.enum.constant_variable.constant  mass=sma_node_mass_kg kg  sp_heat=sma_node_cp J/(K*kg)  mass_min=1e-6 kg  num_ports=foundation.enum.numPorts2.one  m_specify=off  m_priority=High  m=1 kg  m_nominal_specify=off  m_nominal_value=1  m_nominal_unit=kg  T_specify=on  T_priority=High  T=sma_solver_T_init_21_internal(10) K  T_nominal_specify=off  T_nominal_value=1  T_nominal_unit=K  Q_specify=off  Q_priority=None  Q=0 W  Q_nominal_specify=off  Q_nominal_value=1  Q_nominal_unit=W
  NodeMass_11 : fl_lib/Thermal/Thermal Elements/Thermal Mass  mass_type=foundation.enum.constant_variable.constant  mass=sma_node_mass_kg kg  sp_heat=sma_node_cp J/(K*kg)  mass_min=1e-6 kg  num_ports=foundation.enum.numPorts2.one  m_specify=off  m_priority=High  m=1 kg  m_nominal_specify=off  m_nominal_value=1  m_nominal_unit=kg  T_specify=on  T_priority=High  T=sma_solver_T_init_21_internal(11) K  T_nominal_specify=off  T_nominal_value=1  T_nominal_unit=K  Q_specify=off  Q_priority=None  Q=0 W  Q_nominal_specify=off  Q_nominal_value=1  Q_nominal_unit=W
  NodeMass_12 : fl_lib/Thermal/Thermal Elements/Thermal Mass  mass_type=foundation.enum.constant_variable.constant  mass=sma_node_mass_kg kg  sp_heat=sma_node_cp J/(K*kg)  mass_min=1e-6 kg  num_ports=foundation.enum.numPorts2.one  m_specify=off  m_priority=High  m=1 kg  m_nominal_specify=off  m_nominal_value=1  m_nominal_unit=kg  T_specify=on  T_priority=High  T=sma_solver_T_init_21_internal(12) K  T_nominal_specify=off  T_nominal_value=1  T_nominal_unit=K  Q_specify=off  Q_priority=None  Q=0 W  Q_nominal_specify=off  Q_nominal_value=1  Q_nominal_unit=W
  NodeMass_13 : fl_lib/Thermal/Thermal Elements/Thermal Mass  mass_type=foundation.enum.constant_variable.constant  mass=sma_node_mass_kg kg  sp_heat=sma_node_cp J/(K*kg)  mass_min=1e-6 kg  num_ports=foundation.enum.numPorts2.one  m_specify=off  m_priority=High  m=1 kg  m_nominal_specify=off  m_nominal_value=1  m_nominal_unit=kg  T_specify=on  T_priority=High  T=sma_solver_T_init_21_internal(13) K  T_nominal_specify=off  T_nominal_value=1  T_nominal_unit=K  Q_specify=off  Q_priority=None  Q=0 W  Q_nominal_specify=off  Q_nominal_value=1  Q_nominal_unit=W
  NodeMass_14 : fl_lib/Thermal/Thermal Elements/Thermal Mass  mass_type=foundation.enum.constant_variable.constant  mass=sma_node_mass_kg kg  sp_heat=sma_node_cp J/(K*kg)  mass_min=1e-6 kg  num_ports=foundation.enum.numPorts2.one  m_specify=off  m_priority=High  m=1 kg  m_nominal_specify=off  m_nominal_value=1  m_nominal_unit=kg  T_specify=on  T_priority=High  T=sma_solver_T_init_21_internal(14) K  T_nominal_specify=off  T_nominal_value=1  T_nominal_unit=K  Q_specify=off  Q_priority=None  Q=0 W  Q_nominal_specify=off  Q_nominal_value=1  Q_nominal_unit=W
  NodeMass_15 : fl_lib/Thermal/Thermal Elements/Thermal Mass  mass_type=foundation.enum.constant_variable.constant  mass=sma_node_mass_kg kg  sp_heat=sma_node_cp J/(K*kg)  mass_min=1e-6 kg  num_ports=foundation.enum.numPorts2.one  m_specify=off  m_priority=High  m=1 kg  m_nominal_specify=off  m_nominal_value=1  m_nominal_unit=kg  T_specify=on  T_priority=High  T=sma_solver_T_init_21_internal(15) K  T_nominal_specify=off  T_nominal_value=1  T_nominal_unit=K  Q_specify=off  Q_priority=None  Q=0 W  Q_nominal_specify=off  Q_nominal_value=1  Q_nominal_unit=W
  NodeMass_16 : fl_lib/Thermal/Thermal Elements/Thermal Mass  mass_type=foundation.enum.constant_variable.constant  mass=sma_node_mass_kg kg  sp_heat=sma_node_cp J/(K*kg)  mass_min=1e-6 kg  num_ports=foundation.enum.numPorts2.one  m_specify=off  m_priority=High  m=1 kg  m_nominal_specify=off  m_nominal_value=1  m_nominal_unit=kg  T_specify=on  T_priority=High  T=sma_solver_T_init_21_internal(16) K  T_nominal_specify=off  T_nominal_value=1  T_nominal_unit=K  Q_specify=off  Q_priority=None  Q=0 W  Q_nominal_specify=off  Q_nominal_value=1  Q_nominal_unit=W
  NodeMass_17 : fl_lib/Thermal/Thermal Elements/Thermal Mass  mass_type=foundation.enum.constant_variable.constant  mass=sma_node_mass_kg kg  sp_heat=sma_node_cp J/(K*kg)  mass_min=1e-6 kg  num_ports=foundation.enum.numPorts2.one  m_specify=off  m_priority=High  m=1 kg  m_nominal_specify=off  m_nominal_value=1  m_nominal_unit=kg  T_specify=on  T_priority=High  T=sma_solver_T_init_21_internal(17) K  T_nominal_specify=off  T_nominal_value=1  T_nominal_unit=K  Q_specify=off  Q_priority=None  Q=0 W  Q_nominal_specify=off  Q_nominal_value=1  Q_nominal_unit=W
  NodeMass_18 : fl_lib/Thermal/Thermal Elements/Thermal Mass  mass_type=foundation.enum.constant_variable.constant  mass=sma_node_mass_kg kg  sp_heat=sma_node_cp J/(K*kg)  mass_min=1e-6 kg  num_ports=foundation.enum.numPorts2.one  m_specify=off  m_priority=High  m=1 kg  m_nominal_specify=off  m_nominal_value=1  m_nominal_unit=kg  T_specify=on  T_priority=High  T=sma_solver_T_init_21_internal(18) K  T_nominal_specify=off  T_nominal_value=1  T_nominal_unit=K  Q_specify=off  Q_priority=None  Q=0 W  Q_nominal_specify=off  Q_nominal_value=1  Q_nominal_unit=W
  NodeMass_19 : fl_lib/Thermal/Thermal Elements/Thermal Mass  mass_type=foundation.enum.constant_variable.constant  mass=sma_node_mass_kg kg  sp_heat=sma_node_cp J/(K*kg)  mass_min=1e-6 kg  num_ports=foundation.enum.numPorts2.one  m_specify=off  m_priority=High  m=1 kg  m_nominal_specify=off  m_nominal_value=1  m_nominal_unit=kg  T_specify=on  T_priority=High  T=sma_solver_T_init_21_internal(19) K  T_nominal_specify=off  T_nominal_value=1  T_nominal_unit=K  Q_specify=off  Q_priority=None  Q=0 W  Q_nominal_specify=off  Q_nominal_value=1  Q_nominal_unit=W
  NodeMass_20 : fl_lib/Thermal/Thermal Elements/Thermal Mass  mass_type=foundation.enum.constant_variable.constant  mass=sma_node_mass_kg kg  sp_heat=sma_node_cp J/(K*kg)  mass_min=1e-6 kg  num_ports=foundation.enum.numPorts2.one  m_specify=off  m_priority=High  m=1 kg  m_nominal_specify=off  m_nominal_value=1  m_nominal_unit=kg  T_specify=on  T_priority=High  T=sma_solver_T_init_21_internal(20) K  T_nominal_specify=off  T_nominal_value=1  T_nominal_unit=K  Q_specify=off  Q_priority=None  Q=0 W  Q_nominal_specify=off  Q_nominal_value=1  Q_nominal_unit=W
  NodeMass_21 : fl_lib/Thermal/Thermal Elements/Thermal Mass  mass_type=foundation.enum.constant_variable.constant  mass=sma_node_mass_kg kg  sp_heat=sma_node_cp J/(K*kg)  mass_min=1e-6 kg  num_ports=foundation.enum.numPorts2.one  m_specify=off  m_priority=High  m=1 kg  m_nominal_specify=off  m_nominal_value=1  m_nominal_unit=kg  T_specify=on  T_priority=High  T=sma_solver_T_init_21_internal(21) K  T_nominal_specify=off  T_nominal_value=1  T_nominal_unit=K  Q_specify=off  Q_priority=None  Q=0 W  Q_nominal_specify=off  Q_nominal_value=1  Q_nominal_unit=W
  NodeTempPS_01 : nesl_utility/PS-Simulink Converter  PhysicalDomain=network_engine_domain  SubClassName=ps_output  LeftPortType=input  RightPortType=output  PseudoPeriodic=off  Frequencies=[]  VectorFormat=1-D array  Unit=K  AffineConversion=off
  NodeTempPS_02 : nesl_utility/PS-Simulink Converter  PhysicalDomain=network_engine_domain  SubClassName=ps_output  LeftPortType=input  RightPortType=output  PseudoPeriodic=off  Frequencies=[]  VectorFormat=1-D array  Unit=K  AffineConversion=off
  NodeTempPS_03 : nesl_utility/PS-Simulink Converter  PhysicalDomain=network_engine_domain  SubClassName=ps_output  LeftPortType=input  RightPortType=output  PseudoPeriodic=off  Frequencies=[]  VectorFormat=1-D array  Unit=K  AffineConversion=off
  NodeTempPS_04 : nesl_utility/PS-Simulink Converter  PhysicalDomain=network_engine_domain  SubClassName=ps_output  LeftPortType=input  RightPortType=output  PseudoPeriodic=off  Frequencies=[]  VectorFormat=1-D array  Unit=K  AffineConversion=off
  NodeTempPS_05 : nesl_utility/PS-Simulink Converter  PhysicalDomain=network_engine_domain  SubClassName=ps_output  LeftPortType=input  RightPortType=output  PseudoPeriodic=off  Frequencies=[]  VectorFormat=1-D array  Unit=K  AffineConversion=off
  NodeTempPS_06 : nesl_utility/PS-Simulink Converter  PhysicalDomain=network_engine_domain  SubClassName=ps_output  LeftPortType=input  RightPortType=output  PseudoPeriodic=off  Frequencies=[]  VectorFormat=1-D array  Unit=K  AffineConversion=off
  NodeTempPS_07 : nesl_utility/PS-Simulink Converter  PhysicalDomain=network_engine_domain  SubClassName=ps_output  LeftPortType=input  RightPortType=output  PseudoPeriodic=off  Frequencies=[]  VectorFormat=1-D array  Unit=K  AffineConversion=off
  NodeTempPS_08 : nesl_utility/PS-Simulink Converter  PhysicalDomain=network_engine_domain  SubClassName=ps_output  LeftPortType=input  RightPortType=output  PseudoPeriodic=off  Frequencies=[]  VectorFormat=1-D array  Unit=K  AffineConversion=off
  NodeTempPS_09 : nesl_utility/PS-Simulink Converter  PhysicalDomain=network_engine_domain  SubClassName=ps_output  LeftPortType=input  RightPortType=output  PseudoPeriodic=off  Frequencies=[]  VectorFormat=1-D array  Unit=K  AffineConversion=off
  NodeTempPS_{10..21} (12 alike) : nesl_utility/PS-Simulink Converter  PhysicalDomain=network_engine_domain  SubClassName=ps_output  LeftPortType=input  RightPortType=output  PseudoPeriodic=off  Frequencies=[]  VectorFormat=1-D array  Unit=K  AffineConversion=off
  NodeTempSensor_01 : fl_lib/Thermal/Thermal Sensors/Temperature Sensor  temperature_measure=foundation.enum.MeasurementReference.difference
  NodeTempSensor_02 : fl_lib/Thermal/Thermal Sensors/Temperature Sensor  temperature_measure=foundation.enum.MeasurementReference.difference
  NodeTempSensor_03 : fl_lib/Thermal/Thermal Sensors/Temperature Sensor  temperature_measure=foundation.enum.MeasurementReference.difference
  NodeTempSensor_04 : fl_lib/Thermal/Thermal Sensors/Temperature Sensor  temperature_measure=foundation.enum.MeasurementReference.difference
  NodeTempSensor_05 : fl_lib/Thermal/Thermal Sensors/Temperature Sensor  temperature_measure=foundation.enum.MeasurementReference.difference
  NodeTempSensor_06 : fl_lib/Thermal/Thermal Sensors/Temperature Sensor  temperature_measure=foundation.enum.MeasurementReference.difference
  NodeTempSensor_07 : fl_lib/Thermal/Thermal Sensors/Temperature Sensor  temperature_measure=foundation.enum.MeasurementReference.difference
  NodeTempSensor_08 : fl_lib/Thermal/Thermal Sensors/Temperature Sensor  temperature_measure=foundation.enum.MeasurementReference.difference
  NodeTempSensor_09 : fl_lib/Thermal/Thermal Sensors/Temperature Sensor  temperature_measure=foundation.enum.MeasurementReference.difference
  NodeTempSensor_{10..21} (12 alike) : fl_lib/Thermal/Thermal Sensors/Temperature Sensor  temperature_measure=foundation.enum.MeasurementReference.difference
  TempMux51 : Mux  Inputs=21
  ThermalReference51 : fl_lib/Thermal/Thermal Elements/Thermal Reference
  ToWorkspace_Tx21_internal : ToWorkspace  VariableName=SMA_Tx21_internal  SaveFormat=Structure With Time  SampleTime=-1
  Conn1 : PMIOPort  Side=Right
  Conn2 : PMIOPort  Port=2  Side=Right
  Conn3 : PMIOPort  Port=3  Side=Right
  Conn4 : PMIOPort  Port=4  Side=Right
  Conn5 : PMIOPort  Port=5  Side=Right
  Conn6 : PMIOPort  Port=6  Side=Right
  Conn7 : PMIOPort  Port=7  Side=Right
  Conn8 : PMIOPort  Port=8  Side=Right
  Conn9 : PMIOPort  Port=9  Side=Right
  Conn10 : PMIOPort  Port=10  Side=Right
  Conn11 : PMIOPort  Port=11  Side=Right
  Conn12 : PMIOPort  Port=12  Side=Right
  Conn13 : PMIOPort  Port=13  Side=Right
  Conn14 : PMIOPort  Port=14  Side=Right
  Conn15 : PMIOPort  Port=15  Side=Right
  Conn16 : PMIOPort  Port=16  Side=Right
  Conn17 : PMIOPort  Port=17  Side=Right
  Conn18 : PMIOPort  Port=18  Side=Right
  Conn19 : PMIOPort  Port=19  Side=Right
  Conn20 : PMIOPort  Port=20  Side=Right
  Conn21 : PMIOPort  Port=21  Side=Right
  Conn22 : PMIOPort  Port=22  Side=Right
  Conn23 : PMIOPort  Port=23  Side=Right
  Conn24 : PMIOPort  Port=24  Side=Right
  Conn25 : PMIOPort  Port=25  Side=Right
  Conn26 : PMIOPort  Port=26  Side=Right
  Conn27 : PMIOPort  Port=27  Side=Right
  Conn28 : PMIOPort  Port=28  Side=Right
  Conn29 : PMIOPort  Port=29  Side=Right
  Conn30 : PMIOPort  Port=30  Side=Right
  Conn31 : PMIOPort  Port=31  Side=Right
  Conn32 : PMIOPort  Port=32  Side=Right
  Conn33 : PMIOPort  Port=33  Side=Right
  Conn34 : PMIOPort  Port=34  Side=Right
  Conn35 : PMIOPort  Port=35  Side=Right
  Conn36 : PMIOPort  Port=36  Side=Right
  Conn37 : PMIOPort  Port=37  Side=Right
  Conn38 : PMIOPort  Port=38  Side=Right
  Conn39 : PMIOPort  Port=39  Side=Right
  Conn40 : PMIOPort  Port=40  Side=Right
  Conn41 : PMIOPort  Port=41  Side=Right
  Conn42 : PMIOPort  Port=42  Side=Right
  NodeTemp21Out : Outport
  wires:
  NodeTempPS_21/1 -> TempMux51/21
  NodeTempPS_20/1 -> TempMux51/20
  NodeTempPS_19/1 -> TempMux51/19
  NodeTempPS_18/1 -> TempMux51/18
  NodeTempPS_17/1 -> TempMux51/17
  NodeTempPS_16/1 -> TempMux51/16
  NodeTempPS_15/1 -> TempMux51/15
  NodeTempPS_14/1 -> TempMux51/14
  NodeTempPS_13/1 -> TempMux51/13
  NodeTempPS_12/1 -> TempMux51/12
  NodeTempPS_11/1 -> TempMux51/11
  NodeTempPS_10/1 -> TempMux51/10
  NodeTempPS_09/1 -> TempMux51/9
  NodeTempPS_08/1 -> TempMux51/8
  NodeTempPS_07/1 -> TempMux51/7
  NodeTempPS_06/1 -> TempMux51/6
  NodeTempPS_05/1 -> TempMux51/5
  NodeTempPS_04/1 -> TempMux51/4
  NodeTempPS_03/1 -> TempMux51/3
  NodeTempPS_02/1 -> TempMux51/2
  NodeTempPS_01/1 -> TempMux51/1
  TempMux51/1 -> ToWorkspace_Tx21_internal/1, NodeTemp21Out/1
  ConstitutiveHeat21_W/1 -> ConstitutiveHeatDemux21/1
  ConstitutiveHeatDemux21/1 -> ConstitutiveHeatPS_01/1
  ConstitutiveHeatDemux21/2 -> ConstitutiveHeatPS_02/1
  ConstitutiveHeatDemux21/3 -> ConstitutiveHeatPS_03/1
  ConstitutiveHeatDemux21/4 -> ConstitutiveHeatPS_04/1
  ConstitutiveHeatDemux21/5 -> ConstitutiveHeatPS_05/1
  ConstitutiveHeatDemux21/6 -> ConstitutiveHeatPS_06/1
  ConstitutiveHeatDemux21/7 -> ConstitutiveHeatPS_07/1
  ConstitutiveHeatDemux21/8 -> ConstitutiveHeatPS_08/1
  ConstitutiveHeatDemux21/9 -> ConstitutiveHeatPS_09/1
  ConstitutiveHeatDemux21/10 -> ConstitutiveHeatPS_10/1
  ConstitutiveHeatDemux21/11 -> ConstitutiveHeatPS_11/1
  ConstitutiveHeatDemux21/12 -> ConstitutiveHeatPS_12/1
  ConstitutiveHeatDemux21/13 -> ConstitutiveHeatPS_13/1
  ConstitutiveHeatDemux21/14 -> ConstitutiveHeatPS_14/1
  ConstitutiveHeatDemux21/15 -> ConstitutiveHeatPS_15/1
  ConstitutiveHeatDemux21/16 -> ConstitutiveHeatPS_16/1
  ConstitutiveHeatDemux21/17 -> ConstitutiveHeatPS_17/1
  ConstitutiveHeatDemux21/18 -> ConstitutiveHeatPS_18/1
  ConstitutiveHeatDemux21/19 -> ConstitutiveHeatPS_19/1
  ConstitutiveHeatDemux21/20 -> ConstitutiveHeatPS_20/1
  ConstitutiveHeatDemux21/21 -> ConstitutiveHeatPS_21/1
  connections:
  NodeTempSensor_21/RConn2 -- NodeTempPS_21/LConn1
  Conn42/RConn1 -- Conn21/RConn1 -- NodeCond_20_21/RConn1 -- NodeMass_21/LConn1 -- NodeTempSensor_21/LConn1 -- ConstitutiveHeatSource_21/LConn1 -- AxialConduction_020_021/RConn1
  NodeTempSensor_20/RConn2 -- NodeTempPS_20/LConn1
  Conn41/RConn1 -- Conn20/RConn1 -- NodeCond_20_21/LConn1 -- NodeCond_19_20/RConn1 -- NodeMass_20/LConn1 -- NodeTempSensor_20/LConn1 -- ConstitutiveHeatSource_20/LConn1 -- AxialConduction_019_020/RConn1 -- AxialConduction_020_021/LConn1
  NodeTempSensor_19/RConn2 -- NodeTempPS_19/LConn1
  Conn40/RConn1 -- Conn19/RConn1 -- NodeCond_19_20/LConn1 -- NodeCond_18_19/RConn1 -- NodeMass_19/LConn1 -- NodeTempSensor_19/LConn1 -- ConstitutiveHeatSource_19/LConn1 -- AxialConduction_018_019/RConn1 -- AxialConduction_019_020/LConn1
  NodeTempSensor_18/RConn2 -- NodeTempPS_18/LConn1
  Conn39/RConn1 -- Conn18/RConn1 -- NodeCond_18_19/LConn1 -- NodeCond_17_18/RConn1 -- NodeMass_18/LConn1 -- NodeTempSensor_18/LConn1 -- ConstitutiveHeatSource_18/LConn1 -- AxialConduction_017_018/RConn1 -- AxialConduction_018_019/LConn1
  NodeTempSensor_17/RConn2 -- NodeTempPS_17/LConn1
  Conn38/RConn1 -- Conn17/RConn1 -- NodeCond_17_18/LConn1 -- NodeCond_16_17/RConn1 -- NodeMass_17/LConn1 -- NodeTempSensor_17/LConn1 -- ConstitutiveHeatSource_17/LConn1 -- AxialConduction_016_017/RConn1 -- AxialConduction_017_018/LConn1
  NodeTempSensor_16/RConn2 -- NodeTempPS_16/LConn1
  Conn37/RConn1 -- Conn16/RConn1 -- NodeCond_16_17/LConn1 -- NodeCond_15_16/RConn1 -- NodeMass_16/LConn1 -- NodeTempSensor_16/LConn1 -- ConstitutiveHeatSource_16/LConn1 -- AxialConduction_015_016/RConn1 -- AxialConduction_016_017/LConn1
  NodeTempSensor_15/RConn2 -- NodeTempPS_15/LConn1
  Conn36/RConn1 -- Conn15/RConn1 -- NodeCond_15_16/LConn1 -- NodeCond_14_15/RConn1 -- NodeMass_15/LConn1 -- NodeTempSensor_15/LConn1 -- ConstitutiveHeatSource_15/LConn1 -- AxialConduction_014_015/RConn1 -- AxialConduction_015_016/LConn1
  NodeTempSensor_14/RConn2 -- NodeTempPS_14/LConn1
  Conn35/RConn1 -- Conn14/RConn1 -- NodeCond_14_15/LConn1 -- NodeCond_13_14/RConn1 -- NodeMass_14/LConn1 -- NodeTempSensor_14/LConn1 -- ConstitutiveHeatSource_14/LConn1 -- AxialConduction_013_014/RConn1 -- AxialConduction_014_015/LConn1
  NodeTempSensor_13/RConn2 -- NodeTempPS_13/LConn1
  Conn34/RConn1 -- Conn13/RConn1 -- NodeCond_13_14/LConn1 -- NodeCond_12_13/RConn1 -- NodeMass_13/LConn1 -- NodeTempSensor_13/LConn1 -- ConstitutiveHeatSource_13/LConn1 -- AxialConduction_012_013/RConn1 -- AxialConduction_013_014/LConn1
  NodeTempSensor_12/RConn2 -- NodeTempPS_12/LConn1
  Conn33/RConn1 -- Conn12/RConn1 -- NodeCond_12_13/LConn1 -- NodeCond_11_12/RConn1 -- NodeMass_12/LConn1 -- NodeTempSensor_12/LConn1 -- ConstitutiveHeatSource_12/LConn1 -- AxialConduction_011_012/RConn1 -- AxialConduction_012_013/LConn1
  NodeTempSensor_11/RConn2 -- NodeTempPS_11/LConn1
  Conn32/RConn1 -- Conn11/RConn1 -- NodeCond_11_12/LConn1 -- NodeCond_10_11/RConn1 -- NodeMass_11/LConn1 -- NodeTempSensor_11/LConn1 -- ConstitutiveHeatSource_11/LConn1 -- AxialConduction_010_011/RConn1 -- AxialConduction_011_012/LConn1
  NodeTempSensor_10/RConn2 -- NodeTempPS_10/LConn1
  Conn31/RConn1 -- Conn10/RConn1 -- NodeCond_10_11/LConn1 -- NodeCond_09_10/RConn1 -- NodeMass_10/LConn1 -- NodeTempSensor_10/LConn1 -- ConstitutiveHeatSource_10/LConn1 -- AxialConduction_009_010/RConn1 -- AxialConduction_010_011/LConn1
  NodeTempSensor_09/RConn2 -- NodeTempPS_09/LConn1
  Conn30/RConn1 -- Conn9/RConn1 -- NodeCond_09_10/LConn1 -- NodeCond_08_09/RConn1 -- NodeMass_09/LConn1 -- NodeTempSensor_09/LConn1 -- ConstitutiveHeatSource_09/LConn1 -- AxialConduction_008_009/RConn1 -- AxialConduction_009_010/LConn1
  NodeTempSensor_08/RConn2 -- NodeTempPS_08/LConn1
  Conn29/RConn1 -- Conn8/RConn1 -- NodeCond_08_09/LConn1 -- NodeCond_07_08/RConn1 -- NodeMass_08/LConn1 -- NodeTempSensor_08/LConn1 -- ConstitutiveHeatSource_08/LConn1 -- AxialConduction_007_008/RConn1 -- AxialConduction_008_009/LConn1
  NodeTempSensor_07/RConn2 -- NodeTempPS_07/LConn1
  Conn28/RConn1 -- Conn7/RConn1 -- NodeCond_07_08/LConn1 -- NodeCond_06_07/RConn1 -- NodeMass_07/LConn1 -- NodeTempSensor_07/LConn1 -- ConstitutiveHeatSource_07/LConn1 -- AxialConduction_006_007/RConn1 -- AxialConduction_007_008/LConn1
  NodeTempSensor_06/RConn2 -- NodeTempPS_06/LConn1
  Conn27/RConn1 -- Conn6/RConn1 -- NodeCond_06_07/LConn1 -- NodeCond_05_06/RConn1 -- NodeMass_06/LConn1 -- NodeTempSensor_06/LConn1 -- ConstitutiveHeatSource_06/LConn1 -- AxialConduction_005_006/RConn1 -- AxialConduction_006_007/LConn1
  NodeTempSensor_05/RConn2 -- NodeTempPS_05/LConn1
  Conn26/RConn1 -- Conn5/RConn1 -- NodeCond_05_06/LConn1 -- NodeCond_04_05/RConn1 -- NodeMass_05/LConn1 -- NodeTempSensor_05/LConn1 -- ConstitutiveHeatSource_05/LConn1 -- AxialConduction_004_005/RConn1 -- AxialConduction_005_006/LConn1
  NodeTempSensor_04/RConn2 -- NodeTempPS_04/LConn1
  Conn25/RConn1 -- Conn4/RConn1 -- NodeCond_04_05/LConn1 -- NodeCond_03_04/RConn1 -- NodeMass_04/LConn1 -- NodeTempSensor_04/LConn1 -- ConstitutiveHeatSource_04/LConn1 -- AxialConduction_003_004/RConn1 -- AxialConduction_004_005/LConn1
  NodeTempSensor_03/RConn2 -- NodeTempPS_03/LConn1
  Conn24/RConn1 -- Conn3/RConn1 -- NodeCond_03_04/LConn1 -- NodeCond_02_03/RConn1 -- NodeMass_03/LConn1 -- NodeTempSensor_03/LConn1 -- ConstitutiveHeatSource_03/LConn1 -- AxialConduction_002_003/RConn1 -- AxialConduction_003_004/LConn1
  NodeTempSensor_02/RConn2 -- NodeTempPS_02/LConn1
  Conn23/RConn1 -- Conn2/RConn1 -- NodeCond_02_03/LConn1 -- NodeCond_01_02/RConn1 -- NodeMass_02/LConn1 -- NodeTempSensor_02/LConn1 -- ConstitutiveHeatSource_02/LConn1 -- AxialConduction_001_002/RConn1 -- AxialConduction_002_003/LConn1
  NodeTempSensor_01/RConn2 -- NodeTempPS_01/LConn1
  NodeTempSensor_21/RConn1 -- NodeTempSensor_20/RConn1 -- NodeTempSensor_19/RConn1 -- NodeTempSensor_18/RConn1 -- NodeTempSensor_17/RConn1 -- NodeTempSensor_16/RConn1 -- NodeTempSensor_15/RConn1 -- NodeTempSensor_14/RConn1 -- NodeTempSensor_13/RConn1 -- NodeTempSensor_12/RConn1 -- NodeTempSensor_11/RConn1 -- NodeTempSensor_10/RConn1 -- NodeTempSensor_09/RConn1 -- NodeTempSensor_08/RConn1 -- NodeTempSensor_07/RConn1 -- NodeTempSensor_06/RConn1 -- NodeTempSensor_05/RConn1 -- NodeTempSensor_04/RConn1 -- NodeTempSensor_03/RConn1 -- NodeTempSensor_02/RConn1 -- NodeTempSensor_01/RConn1 -- ConstitutiveHeatSource_01/RConn2 -- ConstitutiveHeatSource_02/RConn2 -- ConstitutiveHeatSource_03/RConn2 -- ConstitutiveHeatSource_04/RConn2 -- ConstitutiveHeatSource_05/RConn2 -- ConstitutiveHeatSource_06/RConn2 -- ConstitutiveHeatSource_07/RConn2 -- ConstitutiveHeatSource_08/RConn2 -- ConstitutiveHeatSource_09/RConn2 -- ConstitutiveHeatSource_10/RConn2 -- ConstitutiveHeatSource_11/RConn2 -- ConstitutiveHeatSource_12/RConn2 -- ConstitutiveHeatSource_13/RConn2 -- ConstitutiveHeatSource_14/RConn2 -- ConstitutiveHeatSource_15/RConn2 -- ConstitutiveHeatSource_16/RConn2 -- ConstitutiveHeatSource_17/RConn2 -- ConstitutiveHeatSource_18/RConn2 -- ConstitutiveHeatSource_19/RConn2 -- ConstitutiveHeatSource_20/RConn2 -- ThermalReference51/LConn1 -- ConstitutiveHeatSource_21/RConn2
  Conn22/RConn1 -- Conn1/RConn1 -- NodeCond_01_02/LConn1 -- NodeMass_01/LConn1 -- NodeTempSensor_01/LConn1 -- ConstitutiveHeatSource_01/LConn1 -- AxialConduction_001_002/LConn1
  ConstitutiveHeatPS_01/RConn1 -- ConstitutiveHeatSource_01/RConn1
  ConstitutiveHeatPS_02/RConn1 -- ConstitutiveHeatSource_02/RConn1
  ConstitutiveHeatPS_03/RConn1 -- ConstitutiveHeatSource_03/RConn1
  ConstitutiveHeatPS_04/RConn1 -- ConstitutiveHeatSource_04/RConn1
  ConstitutiveHeatPS_05/RConn1 -- ConstitutiveHeatSource_05/RConn1
  ConstitutiveHeatPS_06/RConn1 -- ConstitutiveHeatSource_06/RConn1
  ConstitutiveHeatPS_07/RConn1 -- ConstitutiveHeatSource_07/RConn1
  ConstitutiveHeatPS_08/RConn1 -- ConstitutiveHeatSource_08/RConn1
  ConstitutiveHeatPS_09/RConn1 -- ConstitutiveHeatSource_09/RConn1
  ConstitutiveHeatPS_10/RConn1 -- ConstitutiveHeatSource_10/RConn1
  ConstitutiveHeatPS_11/RConn1 -- ConstitutiveHeatSource_11/RConn1
  ConstitutiveHeatPS_12/RConn1 -- ConstitutiveHeatSource_12/RConn1
  ConstitutiveHeatPS_13/RConn1 -- ConstitutiveHeatSource_13/RConn1
  ConstitutiveHeatPS_14/RConn1 -- ConstitutiveHeatSource_14/RConn1
  ConstitutiveHeatPS_15/RConn1 -- ConstitutiveHeatSource_15/RConn1
  ConstitutiveHeatPS_16/RConn1 -- ConstitutiveHeatSource_16/RConn1
  ConstitutiveHeatPS_17/RConn1 -- ConstitutiveHeatSource_17/RConn1
  ConstitutiveHeatPS_18/RConn1 -- ConstitutiveHeatSource_18/RConn1
  ConstitutiveHeatPS_19/RConn1 -- ConstitutiveHeatSource_19/RConn1
  ConstitutiveHeatPS_20/RConn1 -- ConstitutiveHeatSource_20/RConn1
  ConstitutiveHeatPS_21/RConn1 -- ConstitutiveHeatSource_21/RConn1
